simulink model "HaulageOptimizedOperationSimulation_Bea"  (R2026a)
settings: Solver=FixedStepDiscrete  FixedStep=1
libraries: simulink x10
settings Model: Creator=chimb  LastModifiedBy=linuxpc

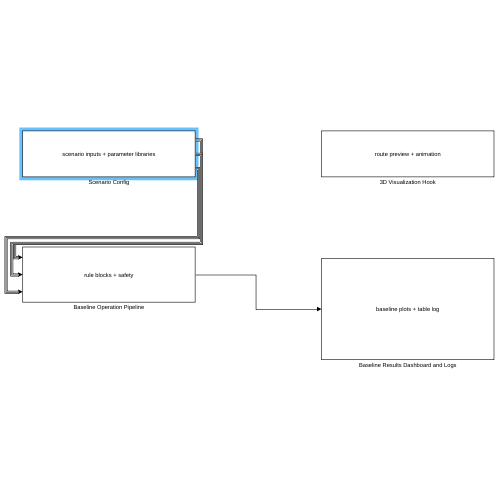
[thumbnail: Simulink's stored preview of the top-level diagram]
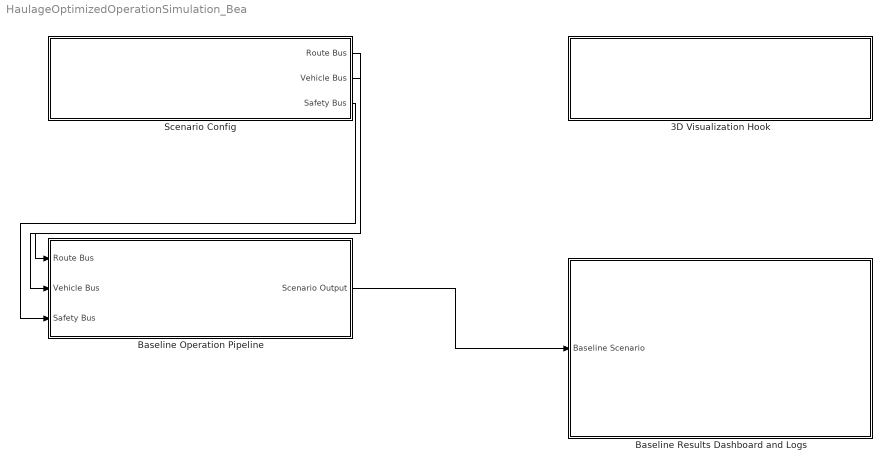
== system HaulageOptimizedOperationSimulation_Bea ==
  3D Visualization Hook : Subsystem
      mask Display: color('black'); disp('route preview + animation')
  Baseline Operation Pipeline : Subsystem
      mask Display: color('black'); disp('rule blocks + safety')
  Baseline Results Dashboard and Logs : Subsystem
      mask Display: color('black'); disp('baseline plots + table log')
  Scenario Config : Subsystem
      mask Display: color('black'); disp('scenario inputs + parameter libraries')
  wires:
  Scenario Config/1(Route Bus) -> Baseline Operation Pipeline/1(Route Bus)
  Scenario Config/2(Vehicle Bus) -> Baseline Operation Pipeline/2(Vehicle Bus)
  Scenario Config/3(Safety Bus) -> Baseline Operation Pipeline/3(Safety Bus)
  Baseline Operation Pipeline/1(Scenario Output) -> Baseline Results Dashboard and Logs/1(Baseline Scenario)

== system HaulageOptimizedOperationSimulation_Bea/3D Visualization Hook ==
  Route 3D Preview Image : Subsystem
      settings: OpenFcn=open('C:/Users/chimb/Documents/Codex/2026-05-20/files-mentioned-by-the-user-paper/haulage_sim_framework/outputs/baseline_operation_route_3d_preview.png')
      mask Display: image(imread('C:/Users/chimb/Documents/Codex/2026-05-20/files-mentioned-by-the-user-paper/haulage_sim_framework/outputs/baseline_operation_route_3d_preview.png'))

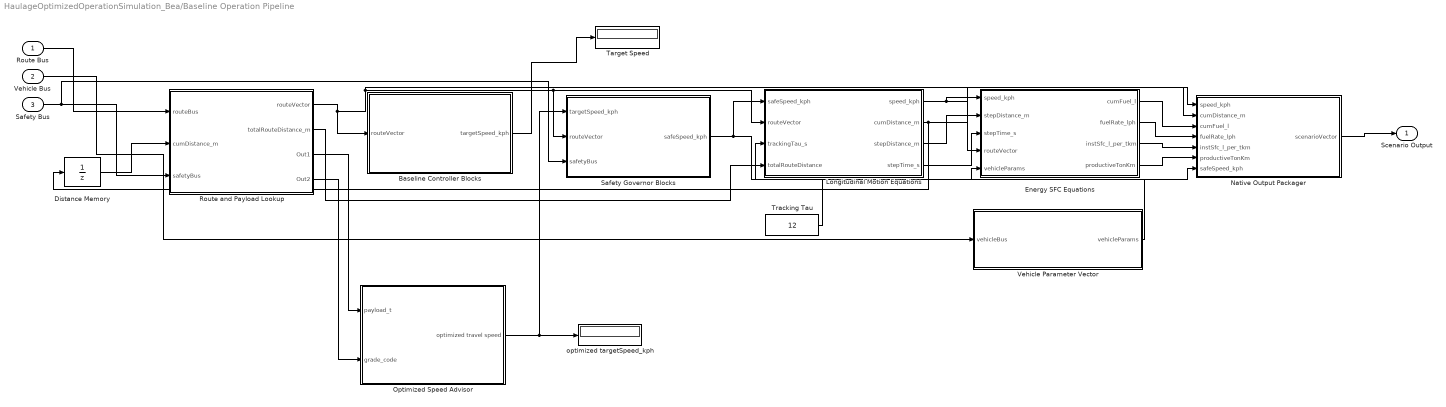
== system HaulageOptimizedOperationSimulation_Bea/Baseline Operation Pipeline ==
  Route Bus : Inport
  Vehicle Bus : Inport  Port=2
  Safety Bus : Inport  Port=3
  Baseline Controller Blocks : Subsystem
      mask Display: color('black'); disp('rule-based speed logic')
  Distance Memory : UnitDelay
  Energy SFC Equations : MATLAB Function  TreatAsAtomicUnit=on
  Longitudinal Motion Equations : MATLAB Function  TreatAsAtomicUnit=on
  Native Output Packager : Subsystem
      mask Display: color('black'); disp('native mux for log vector')
  Optimized Speed Advisor : Subsystem
  Route and Payload Lookup : Subsystem
      mask Display: color('black'); disp('dynamic route lookup tables')
  Safety Governor Blocks : Subsystem
      mask Display: color('black'); disp('speed caps + min/max')
  Target Speed : Display
  Tracking Tau : Constant  Value=12
  Vehicle Parameter Vector : Subsystem
  optimized targetSpeed_kph : Display
  Scenario Output : Outport
  wires:
  Route Bus/1 -> Route and Payload Lookup/1(routeBus)
  Vehicle Bus/1 -> Vehicle Parameter Vector/1(vehicleBus)
  Safety Bus/1 -> Safety Governor Blocks/3(safetyBus), Route and Payload Lookup/3(safetyBus)
  Distance Memory/1 -> Route and Payload Lookup/2(cumDistance_m)
  Route and Payload Lookup/1(routeVector) -> Safety Governor Blocks/2(routeVector), Longitudinal Motion Equations/2(routeVector), Energy SFC Equations/4(routeVector), Baseline Controller Blocks/1(routeVector)
  Baseline Controller Blocks/1(targetSpeed_kph) -> Target Speed/1
  Safety Governor Blocks/1(safeSpeed_kph) -> Longitudinal Motion Equations/1(safeSpeed_kph), Native Output Packager/7(safeSpeed_kph)
  Tracking Tau/1 -> Longitudinal Motion Equations/3(trackingTau_s)
  Route and Payload Lookup/2(totalRouteDistance_m) -> Longitudinal Motion Equations/4(totalRouteDistance)
  Longitudinal Motion Equations/1(speed_kph) -> Energy SFC Equations/1(speed_kph), Native Output Packager/1(speed_kph)
  Longitudinal Motion Equations/3(stepDistance_m) -> Energy SFC Equations/2(stepDistance_m)
  Longitudinal Motion Equations/4(stepTime_s) -> Energy SFC Equations/3(stepTime_s)
  Vehicle Parameter Vector/1(vehicleParams) -> Energy SFC Equations/5(vehicleParams)
  Longitudinal Motion Equations/2(cumDistance_m) -> Native Output Packager/2(cumDistance_m), Distance Memory/1
  Energy SFC Equations/1(cumFuel_l) -> Native Output Packager/3(cumFuel_l)
  Energy SFC Equations/2(fuelRate_lph) -> Native Output Packager/4(fuelRate_lph)
  Energy SFC Equations/3(instSfc_l_per_tkm) -> Native Output Packager/5(instSfc_l_per_tkm)
  Energy SFC Equations/4(productiveTonKm) -> Native Output Packager/6(productiveTonKm)
  Native Output Packager/1(scenarioVector) -> Scenario Output/1
  Route and Payload Lookup/3(Out1) -> Optimized Speed Advisor/1(payload_t)
  Route and Payload Lookup/4(Out2) -> Optimized Speed Advisor/2(grade_code)
  Optimized Speed Advisor/1(optimized travel speed) -> optimized targetSpeed_kph/1, Safety Governor Blocks/1(targetSpeed_kph)

== system HaulageOptimizedOperationSimulation_Bea/Baseline Results Dashboard and Logs ==
  Baseline Scenario : Inport
  Baseline Log : ToWorkspace  VariableName=optimized_operation_log  SaveFormat=Structure With Time  SampleTime=-1
  Baseline Metric Dashboard : Subsystem
      mask Display: color('black'); disp('baseline speed, fuel, SFC, productivity')
  To Workspace : ToWorkspace  VariableName=simout  SaveFormat=Timeseries  SampleTime=-1
  wires:
  Baseline Scenario/1 -> Baseline Log/1, To Workspace/1, Baseline Metric Dashboard/1(Baseline Scenario Vector)

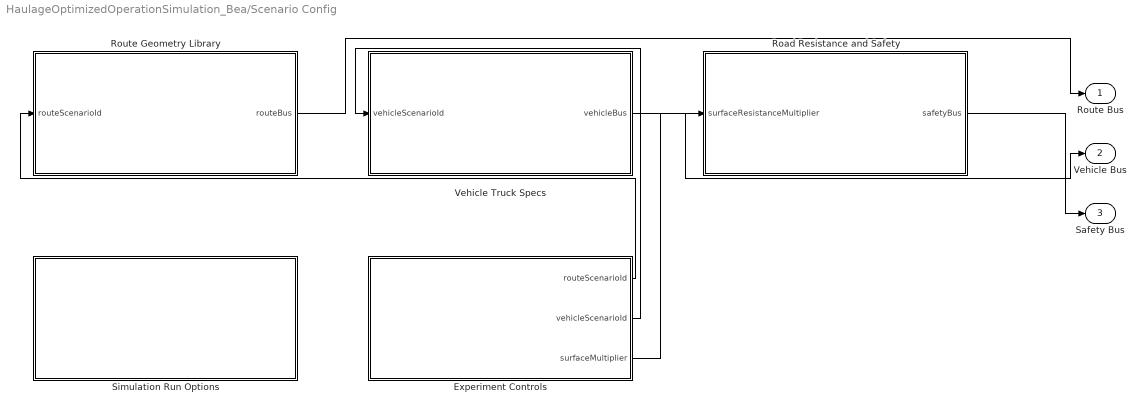
== system HaulageOptimizedOperationSimulation_Bea/Scenario Config ==
  Experiment Controls : Subsystem
      mask Display: color('black'); disp('active experiment selectors')
  Road Resistance and Safety : Subsystem
      mask Display: color('black'); disp('rolling resistance + safety caps')
  Route Geometry Library : Subsystem
      mask Display: color('black'); disp('route segments, grade, limits')
  Simulation Run Options : Subsystem
      mask Display: color('black'); disp('solver, stop time, reporting')
  Vehicle Truck Specs : Subsystem
      mask Display: color('black'); disp('full-scale haul truck specs')
  Route Bus : Outport
  Vehicle Bus : Outport  Port=2
  Safety Bus : Outport  Port=3
  wires:
  Experiment Controls/1(routeScenarioId) -> Route Geometry Library/1(routeScenarioId)
  Experiment Controls/2(vehicleScenarioId) -> Vehicle Truck Specs/1(vehicleScenarioId)
  Experiment Controls/3(surfaceMultiplier) -> Road Resistance and Safety/1(surfaceResistanceMultiplier)
  Route Geometry Library/1(routeBus) -> Route Bus/1
  Vehicle Truck Specs/1(vehicleBus) -> Vehicle Bus/1
  Road Resistance and Safety/1(safetyBus) -> Safety Bus/1

== system HaulageOptimizedOperationSimulation_Bea/3D Visualization Hook/Route 3D Preview Image ==
  Preview Ready Flag : Constant
  Preview Status Display : Display
  wires:
  Preview Ready Flag/1 -> Preview Status Display/1

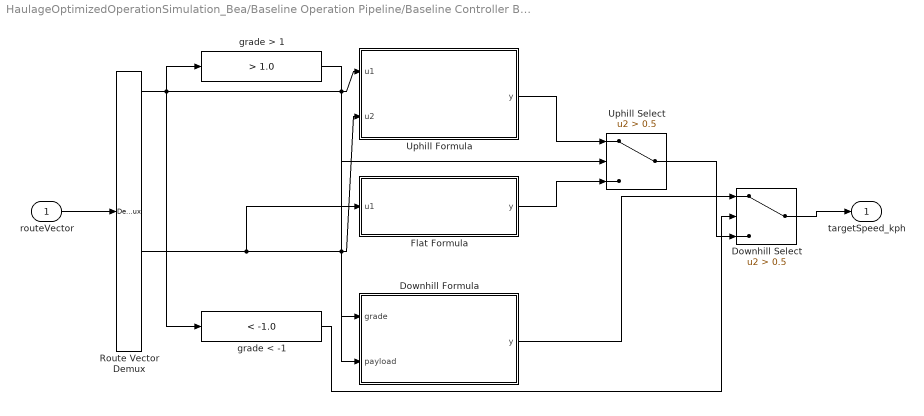
== system HaulageOptimizedOperationSimulation_Bea/Baseline Operation Pipeline/Baseline Controller Blocks ==
  routeVector : Inport
  Downhill Formula : Subsystem
  Downhill Select : Switch  Criteria=u2 > Threshold  Threshold=0.5  SaturateOnIntegerOverflow=off  InputSameDT=off
  Flat Formula : Subsystem
  Route Vector Demux : Demux  Outputs=7
  Uphill Formula : Subsystem
  Uphill Select : Switch  Criteria=u2 > Threshold  Threshold=0.5  SaturateOnIntegerOverflow=off  InputSameDT=off
  grade < -1 : simulink/Logic and Bit Operations/Compare To Constant  relop=<  const=-1.0  OutDataTypeStr=boolean
  grade > 1 : simulink/Logic and Bit Operations/Compare To Constant  relop=>  const=1.0  OutDataTypeStr=boolean
  targetSpeed_kph : Outport
  wires:
  routeVector/1 -> Route Vector Demux/1
  Route Vector Demux/1 -> Uphill Formula/1(u1), Downhill Formula/1(grade), grade > 1/1, grade < -1/1
  Route Vector Demux/5 -> Uphill Formula/2(u2), Downhill Formula/2(payload), Flat Formula/1(u1)
  Uphill Formula/1(y) -> Uphill Select/1
  grade > 1/1 -> Uphill Select/2
  Flat Formula/1(y) -> Uphill Select/3
  Downhill Formula/1(y) -> Downhill Select/1
  grade < -1/1 -> Downhill Select/2
  Uphill Select/1 -> Downhill Select/3
  Downhill Select/1 -> targetSpeed_kph/1

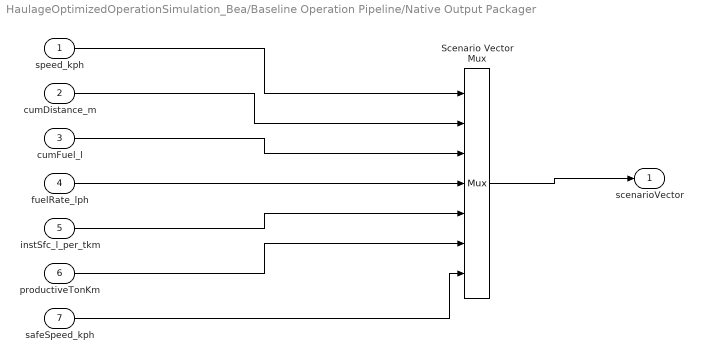
== system HaulageOptimizedOperationSimulation_Bea/Baseline Operation Pipeline/Native Output Packager ==
  speed_kph : Inport
  cumDistance_m : Inport  Port=2
  cumFuel_l : Inport  Port=3
  fuelRate_lph : Inport  Port=4
  instSfc_l_per_tkm : Inport  Port=5
  productiveTonKm : Inport  Port=6
  safeSpeed_kph : Inport  Port=7
  Scenario Vector Mux : Mux  Inputs=7
  scenarioVector : Outport
  wires:
  speed_kph/1 -> Scenario Vector Mux/1
  cumDistance_m/1 -> Scenario Vector Mux/2
  cumFuel_l/1 -> Scenario Vector Mux/3
  fuelRate_lph/1 -> Scenario Vector Mux/4
  instSfc_l_per_tkm/1 -> Scenario Vector Mux/5
  productiveTonKm/1 -> Scenario Vector Mux/6
  safeSpeed_kph/1 -> Scenario Vector Mux/7
  Scenario Vector Mux/1 -> scenarioVector/1

== system HaulageOptimizedOperationSimulation_Bea/Baseline Operation Pipeline/Optimized Speed Advisor ==
  note: opt_speed_kph column from the ml_speed_policy_table.csv
      | For our current open-pit route, the truck is:
      | loaded at 279 t on segments S1-S5;
      | empty at 0 t on segments S6-S8.
  payload_t : Inport
  grade_code : Inport  Port=2
  Downhill : MATLAB Function  TreatAsAtomicUnit=on
  Flat : MATLAB Function  TreatAsAtomicUnit=on
  Multiport Switch : MultiPortSwitch  SaturateOnIntegerOverflow=off  InputSameDT=off
  Uphill : MATLAB Function  TreatAsAtomicUnit=on
  optimized travel speed : Outport
  wires:
  payload_t/1 -> Downhill/1(u), Flat/1(u), Uphill/1(u)
  Uphill/1(y) -> Multiport Switch/2
  Flat/1(y) -> Multiport Switch/3
  Downhill/1(y) -> Multiport Switch/4
  grade_code/1 -> Multiport Switch/1
  Multiport Switch/1 -> optimized travel speed/1

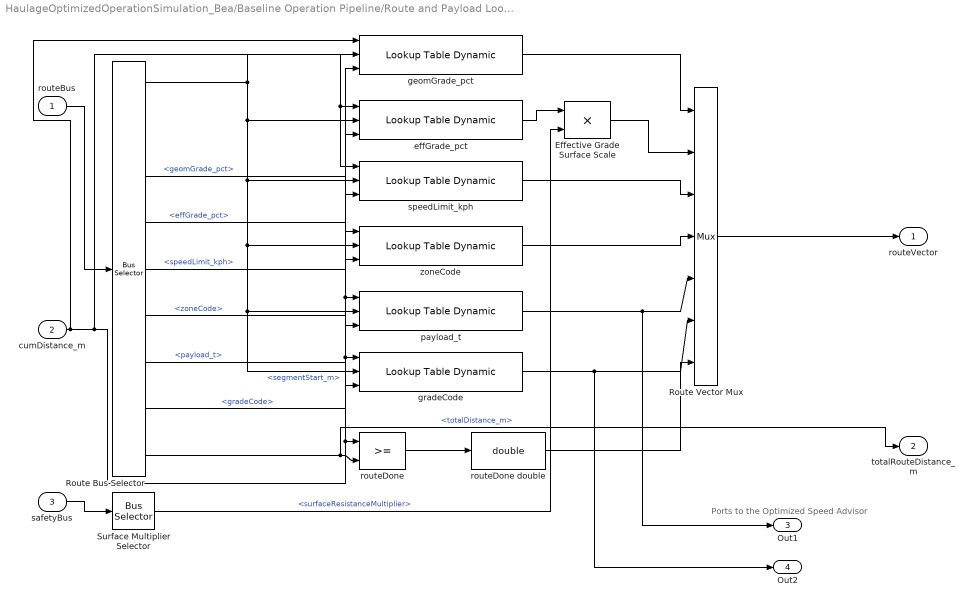
== system HaulageOptimizedOperationSimulation_Bea/Baseline Operation Pipeline/Route and Payload Lookup ==
  note: Ports to the Optimized Speed Advisor
  routeBus : Inport
  cumDistance_m : Inport  Port=2
  safetyBus : Inport  Port=3
  Effective Grade Surface Scale : Product
  Route Bus Selector : BusSelector  OutputSignals=segmentStart_m,segmentEnd_m,geomGrade_pct,effGrade_pct,speedLimit_kph,zoneCode,payload_t,gradeCode,totalDistance_m
  Route Vector Mux : Mux  Inputs=7
  Surface Multiplier Selector : BusSelector  OutputSignals=surfaceResistanceMultiplier
  effGrade_pct : simulink/Lookup Tables/Lookup Table Dynamic  LookUpMeth=Use Input Below  OutDataType=fixdt('double')  OutScaling=[]  OutputDataTypeScalingMode=Specify via dialog  OutDataTypeStr=double  DoSatur=off
  geomGrade_pct : simulink/Lookup Tables/Lookup Table Dynamic  LookUpMeth=Use Input Below  OutDataType=fixdt('double')  OutScaling=[]  OutputDataTypeScalingMode=Specify via dialog  OutDataTypeStr=double  DoSatur=off
  gradeCode : simulink/Lookup Tables/Lookup Table Dynamic  LookUpMeth=Use Input Below  OutDataType=fixdt('double')  OutScaling=[]  OutputDataTypeScalingMode=Specify via dialog  OutDataTypeStr=double  DoSatur=off
  payload_t : simulink/Lookup Tables/Lookup Table Dynamic  LookUpMeth=Use Input Below  OutDataType=fixdt('double')  OutScaling=[]  OutputDataTypeScalingMode=Specify via dialog  OutDataTypeStr=double  DoSatur=off
  routeDone : RelationalOperator  OutDataTypeStr=boolean  RndMeth=Simplest  InputSameDT=off
  routeDone double : DataTypeConversion  OutDataTypeStr=double  SaturateOnIntegerOverflow=off  RndMeth=Floor
  speedLimit_kph : simulink/Lookup Tables/Lookup Table Dynamic  LookUpMeth=Use Input Below  OutDataType=fixdt('double')  OutScaling=[]  OutputDataTypeScalingMode=Specify via dialog  OutDataTypeStr=double  DoSatur=off
  zoneCode : simulink/Lookup Tables/Lookup Table Dynamic  LookUpMeth=Use Input Below  OutDataType=fixdt('double')  OutScaling=[]  OutputDataTypeScalingMode=Specify via dialog  OutDataTypeStr=double  DoSatur=off
  routeVector : Outport
  totalRouteDistance_m : Outport  Port=2
  Out1 : Outport  Port=3
  Out2 : Outport  Port=4
  wires:
  routeBus/1 -> Route Bus Selector/1
  safetyBus/1 -> Surface Multiplier Selector/1
  cumDistance_m/1 -> zoneCode/1, payload_t/1, gradeCode/1, routeDone/1, effGrade_pct/1, speedLimit_kph/1, geomGrade_pct/1
  Route Bus Selector/1 -> payload_t/2, gradeCode/2, zoneCode/2, speedLimit_kph/2, effGrade_pct/2, geomGrade_pct/2  "<segmentStart_m>"
  Route Bus Selector/3 -> geomGrade_pct/3  "<geomGrade_pct>"
  Route Bus Selector/4 -> effGrade_pct/3  "<effGrade_pct>"
  Route Bus Selector/5 -> speedLimit_kph/3  "<speedLimit_kph>"
  Route Bus Selector/6 -> zoneCode/3  "<zoneCode>"
  Route Bus Selector/7 -> payload_t/3  "<payload_t>"
  Route Bus Selector/8 -> gradeCode/3  "<gradeCode>"
  effGrade_pct/1 -> Effective Grade Surface Scale/1
  Surface Multiplier Selector/1 -> Effective Grade Surface Scale/2  "<surfaceResistanceMultiplier>"
  Route Bus Selector/9 -> routeDone/2, totalRouteDistance_m/1  "<totalDistance_m>"
  routeDone/1 -> routeDone double/1
  geomGrade_pct/1 -> Route Vector Mux/1
  Effective Grade Surface Scale/1 -> Route Vector Mux/2
  speedLimit_kph/1 -> Route Vector Mux/3
  zoneCode/1 -> Route Vector Mux/4
  gradeCode/1 -> Out2/1, Route Vector Mux/6
  routeDone double/1 -> Route Vector Mux/7
  Route Vector Mux/1 -> routeVector/1
  payload_t/1 -> Out1/1, Route Vector Mux/5

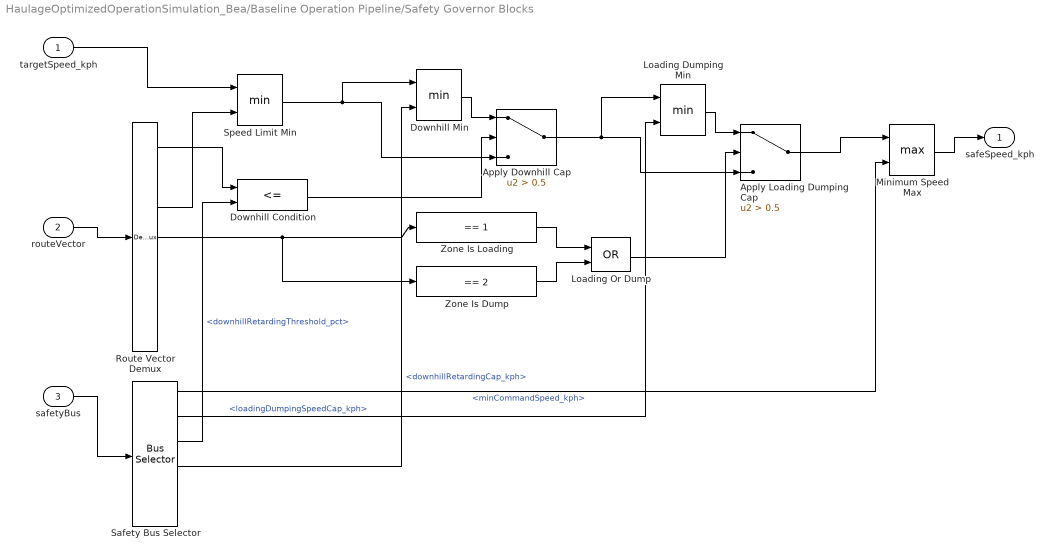
== system HaulageOptimizedOperationSimulation_Bea/Baseline Operation Pipeline/Safety Governor Blocks ==
  targetSpeed_kph : Inport
  routeVector : Inport  Port=2
  safetyBus : Inport  Port=3
  Apply Downhill Cap : Switch  Criteria=u2 > Threshold  Threshold=0.5  SaturateOnIntegerOverflow=off  InputSameDT=off
  Apply Loading Dumping Cap : Switch  Criteria=u2 > Threshold  Threshold=0.5  SaturateOnIntegerOverflow=off  InputSameDT=off
  Downhill Condition : RelationalOperator  Operator=<=  OutDataTypeStr=boolean  RndMeth=Simplest  InputSameDT=off
  Downhill Min : MinMax  Inputs=2
  Loading Dumping Min : MinMax  Inputs=2
  Loading Or Dump : Logic  Operator=OR  AllPortsSameDT=off  OutDataTypeStr=boolean
  Minimum Speed Max : MinMax  Function=max  Inputs=2
  Route Vector Demux : Demux  Outputs=7
  Safety Bus Selector : BusSelector  OutputSignals=minCommandSpeed_kph,loadingDumpingSpeedCap_kph,downhillRetardingThreshold_pct,downhillRetardingCap_kph,maxOperatingSpeed_kph,surfaceResistanceMultiplier
  Speed Limit Min : MinMax  Inputs=2
  Zone Is Dump : simulink/Logic and Bit Operations/Compare To Constant  relop===  const=2  OutDataTypeStr=boolean
  Zone Is Loading : simulink/Logic and Bit Operations/Compare To Constant  relop===  const=1  OutDataTypeStr=boolean
  safeSpeed_kph : Outport
  wires:
  routeVector/1 -> Route Vector Demux/1
  safetyBus/1 -> Safety Bus Selector/1
  targetSpeed_kph/1 -> Speed Limit Min/1
  Route Vector Demux/3 -> Speed Limit Min/2
  Route Vector Demux/1 -> Downhill Condition/1
  Safety Bus Selector/3 -> Downhill Condition/2  "<downhillRetardingThreshold_pct>"
  Speed Limit Min/1 -> Downhill Min/1, Apply Downhill Cap/3
  Safety Bus Selector/4 -> Downhill Min/2  "<downhillRetardingCap_kph>"
  Downhill Min/1 -> Apply Downhill Cap/1
  Downhill Condition/1 -> Apply Downhill Cap/2
  Route Vector Demux/4 -> Zone Is Loading/1, Zone Is Dump/1
  Zone Is Loading/1 -> Loading Or Dump/1
  Zone Is Dump/1 -> Loading Or Dump/2
  Apply Downhill Cap/1 -> Loading Dumping Min/1, Apply Loading Dumping Cap/3
  Safety Bus Selector/2 -> Loading Dumping Min/2  "<loadingDumpingSpeedCap_kph>"
  Loading Dumping Min/1 -> Apply Loading Dumping Cap/1
  Loading Or Dump/1 -> Apply Loading Dumping Cap/2
  Apply Loading Dumping Cap/1 -> Minimum Speed Max/1
  Safety Bus Selector/1 -> Minimum Speed Max/2  "<minCommandSpeed_kph>"
  Minimum Speed Max/1 -> safeSpeed_kph/1

== system HaulageOptimizedOperationSimulation_Bea/Baseline Operation Pipeline/Vehicle Parameter Vector ==
  vehicleBus : Inport
  Vehicle Bus Selector : BusSelector  OutputSignals=emptyMass_kg,idleFuelRate_lph,maxFuelRate_lph,frontalArea_m2,dragCoefficient,drivetrainEfficiency
  Vehicle Params Mux : Mux  Inputs=6
  vehicleParams : Outport
  wires:
  vehicleBus/1 -> Vehicle Bus Selector/1
  Vehicle Bus Selector/1 -> Vehicle Params Mux/1  "<emptyMass_kg>"
  Vehicle Bus Selector/2 -> Vehicle Params Mux/2  "<idleFuelRate_lph>"
  Vehicle Bus Selector/3 -> Vehicle Params Mux/3  "<maxFuelRate_lph>"
  Vehicle Bus Selector/4 -> Vehicle Params Mux/4  "<frontalArea_m2>"
  Vehicle Bus Selector/5 -> Vehicle Params Mux/5  "<dragCoefficient>"
  Vehicle Bus Selector/6 -> Vehicle Params Mux/6  "<drivetrainEfficiency>"
  Vehicle Params Mux/1 -> vehicleParams/1

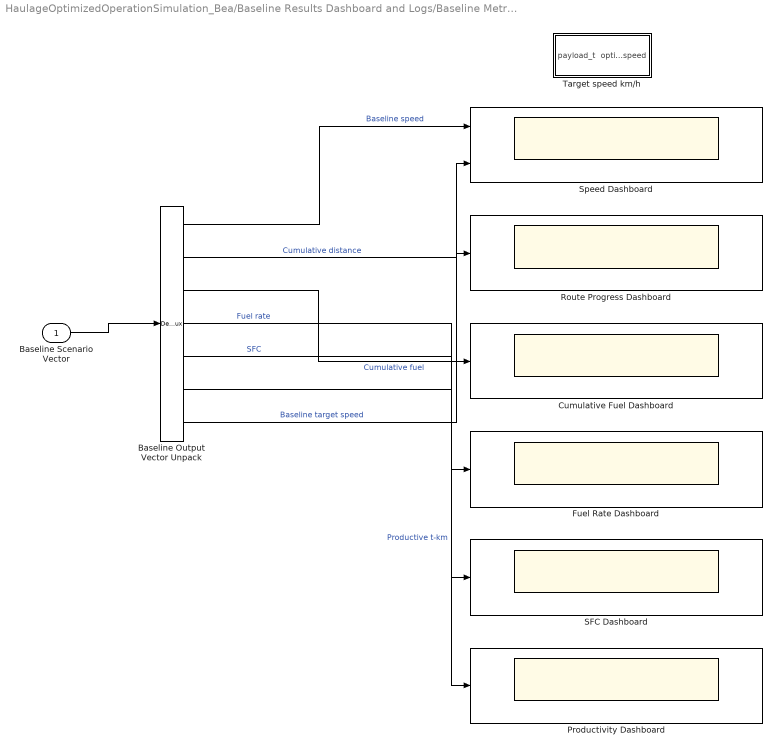
== system HaulageOptimizedOperationSimulation_Bea/Baseline Results Dashboard and Logs/Baseline Metric Dashboard ==
  Baseline Scenario Vector : Inport
  Baseline Output Vector Unpack : Demux  Outputs=7
  Cumulative Fuel Dashboard : Scope
      settings: Title=Baseline Cumulative Fuel Use  ActiveDisplayYMinimum=-0.7369719012317395  ActiveDisplayYMaximum=6.6567683881931847  YLabel=Fuel (L)
  Fuel Rate Dashboard : Scope
      settings: Title=Baseline Fuel Rate Along Cycle  ActiveDisplayYMinimum=-3.9999999999999982  ActiveDisplayYMaximum=106  YLabel=Fuel rate (L/h)
  Productivity Dashboard : Scope
      settings: Title=Baseline Productive Haulage Work  ActiveDisplayYMinimum=-27.831999586920773  ActiveDisplayYMaximum=251.262996282287  YLabel=Productive work (t-km)
  Route Progress Dashboard : Scope
      settings: Title=Baseline Route Progress  ActiveDisplayYMinimum=-192.18749999999994  ActiveDisplayYMaximum=1732.4652777777778  YLabel=Cumulative distance (m)
  SFC Dashboard : Scope
      settings: Title=Baseline Specific Fuel Consumption  ActiveDisplayYMinimum=-0.00247472099881277  ActiveDisplayYMaximum=0.036217610604932046  YLabel=SFC (L/t-km)
  Speed Dashboard : Scope  NumInputPorts=2
      settings: Title=Baseline Speed and Command  ActiveDisplayYMinimum=-1.1249999999999998  ActiveDisplayYMaximum=20.125  YLabel=Speed (km/h)
  Target speed km/h : Subsystem
  wires:
  Baseline Scenario Vector/1 -> Baseline Output Vector Unpack/1
  Baseline Output Vector Unpack/1 -> Speed Dashboard/1  "Baseline speed"
  Baseline Output Vector Unpack/7 -> Speed Dashboard/2  "Baseline target speed"
  Baseline Output Vector Unpack/2 -> Route Progress Dashboard/1  "Cumulative distance"
  Baseline Output Vector Unpack/3 -> Cumulative Fuel Dashboard/1  "Cumulative fuel"
  Baseline Output Vector Unpack/4 -> Fuel Rate Dashboard/1  "Fuel rate"
  Baseline Output Vector Unpack/5 -> SFC Dashboard/1  "SFC"
  Baseline Output Vector Unpack/6 -> Productivity Dashboard/1  "Productive t-km"

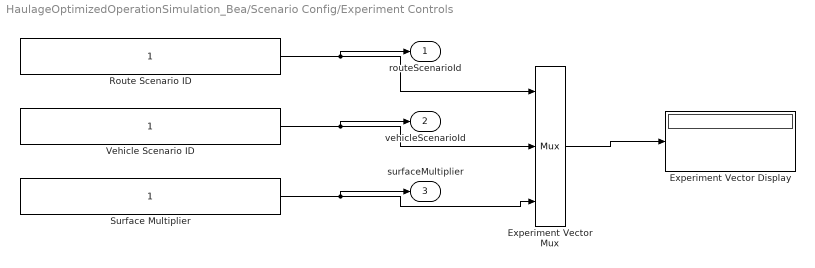
== system HaulageOptimizedOperationSimulation_Bea/Scenario Config/Experiment Controls ==
  Experiment Vector Display : Display
  Experiment Vector Mux : Mux  Inputs=3
  Route Scenario ID : Constant
  Surface Multiplier : Constant
  Vehicle Scenario ID : Constant
  routeScenarioId : Outport
  vehicleScenarioId : Outport  Port=2
  surfaceMultiplier : Outport  Port=3
  wires:
  Route Scenario ID/1 -> Experiment Vector Mux/1, routeScenarioId/1
  Vehicle Scenario ID/1 -> Experiment Vector Mux/2, vehicleScenarioId/1
  Surface Multiplier/1 -> Experiment Vector Mux/3, surfaceMultiplier/1
  Experiment Vector Mux/1 -> Experiment Vector Display/1

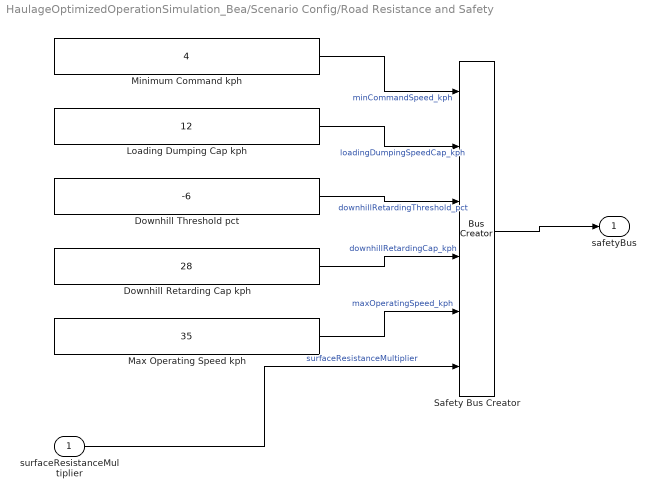
== system HaulageOptimizedOperationSimulation_Bea/Scenario Config/Road Resistance and Safety ==
  surfaceResistanceMultiplier : Inport
  Downhill Retarding Cap kph : Constant  Value=28
  Downhill Threshold pct : Constant  Value=-6
  Loading Dumping Cap kph : Constant  Value=12
  Max Operating Speed kph : Constant  Value=35
  Minimum Command kph : Constant  Value=4
  Safety Bus Creator : BusCreator  Inputs=6
  safetyBus : Outport
  wires:
  Minimum Command kph/1 -> Safety Bus Creator/1  "minCommandSpeed_kph"
  Loading Dumping Cap kph/1 -> Safety Bus Creator/2  "loadingDumpingSpeedCap_kph"
  Downhill Threshold pct/1 -> Safety Bus Creator/3  "downhillRetardingThreshold_pct"
  Downhill Retarding Cap kph/1 -> Safety Bus Creator/4  "downhillRetardingCap_kph"
  Max Operating Speed kph/1 -> Safety Bus Creator/5  "maxOperatingSpeed_kph"
  surfaceResistanceMultiplier/1 -> Safety Bus Creator/6  "surfaceResistanceMultiplier"
  Safety Bus Creator/1 -> safetyBus/1

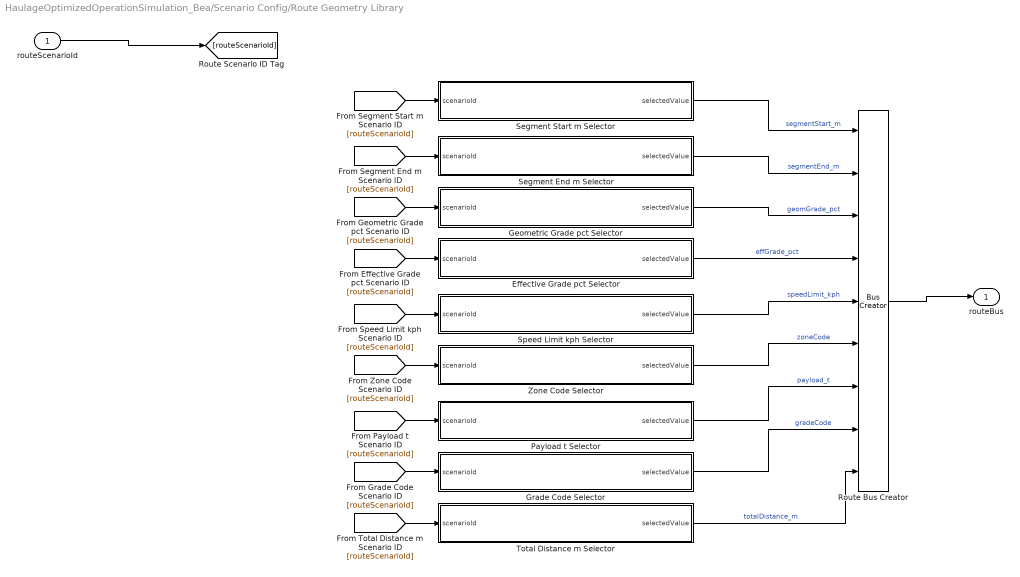
== system HaulageOptimizedOperationSimulation_Bea/Scenario Config/Route Geometry Library ==
  routeScenarioId : Inport
  Effective Grade pct Selector : Subsystem
      mask Display: color('black'); disp('editable effective grade pct scenario selector')
  Geometric Grade pct Selector : Subsystem
      mask Display: color('black'); disp('editable geometric grade pct scenario selector')
  Grade Code Selector : Subsystem
      mask Display: color('black'); disp('editable grade code scenario selector')
  Payload t Selector : Subsystem
      mask Display: color('black'); disp('editable payload t scenario selector')
  Route Bus Creator : BusCreator  Inputs=9
  Segment End m Selector : Subsystem
      mask Display: color('black'); disp('editable segment end m scenario selector')
  Segment Start m Selector : Subsystem
      mask Display: color('black'); disp('editable segment start m scenario selector')
  Speed Limit kph Selector : Subsystem
      mask Display: color('black'); disp('editable speed limit kph scenario selector')
  Total Distance m Selector : Subsystem
      mask Display: color('black'); disp('editable total distance m scenario selector')
  Zone Code Selector : Subsystem
      mask Display: color('black'); disp('editable zone code scenario selector')
  routeBus : Outport
  wires:
  routeScenarioId/1 -> [routeScenarioId]
  [routeScenarioId] -> Segment Start m Selector/1(scenarioId)
  [routeScenarioId] -> Segment End m Selector/1(scenarioId)
  [routeScenarioId] -> Geometric Grade pct Selector/1(scenarioId)
  [routeScenarioId] -> Effective Grade pct Selector/1(scenarioId)
  [routeScenarioId] -> Speed Limit kph Selector/1(scenarioId)
  [routeScenarioId] -> Zone Code Selector/1(scenarioId)
  [routeScenarioId] -> Payload t Selector/1(scenarioId)
  [routeScenarioId] -> Grade Code Selector/1(scenarioId)
  [routeScenarioId] -> Total Distance m Selector/1(scenarioId)
  Segment Start m Selector/1(selectedValue) -> Route Bus Creator/1  "segmentStart_m"
  Segment End m Selector/1(selectedValue) -> Route Bus Creator/2  "segmentEnd_m"
  Geometric Grade pct Selector/1(selectedValue) -> Route Bus Creator/3  "geomGrade_pct"
  Effective Grade pct Selector/1(selectedValue) -> Route Bus Creator/4  "effGrade_pct"
  Speed Limit kph Selector/1(selectedValue) -> Route Bus Creator/5  "speedLimit_kph"
  Zone Code Selector/1(selectedValue) -> Route Bus Creator/6  "zoneCode"
  Payload t Selector/1(selectedValue) -> Route Bus Creator/7  "payload_t"
  Grade Code Selector/1(selectedValue) -> Route Bus Creator/8  "gradeCode"
  Total Distance m Selector/1(selectedValue) -> Route Bus Creator/9  "totalDistance_m"
  Route Bus Creator/1 -> routeBus/1

== system HaulageOptimizedOperationSimulation_Bea/Scenario Config/Simulation Run Options ==
  Baseline Tracking Tau s : Constant  Value=12
  Clock Display : Display
  Fixed Step dt s : Constant
  Output Vector Width : Constant  Value=7
  Simulation Clock : Clock
  Stop Time s : Constant  Value=1400
  wires:
  Simulation Clock/1 -> Clock Display/1

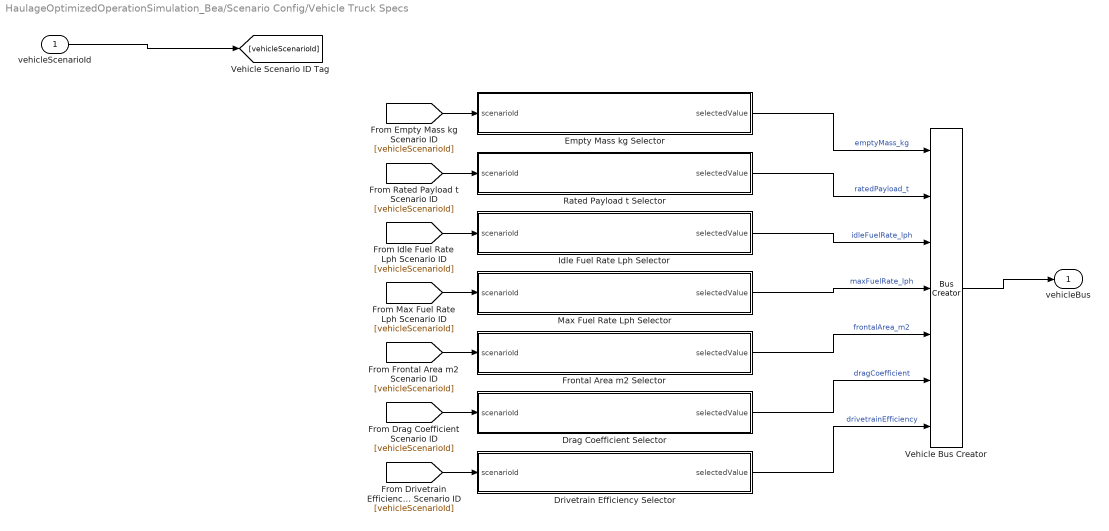
== system HaulageOptimizedOperationSimulation_Bea/Scenario Config/Vehicle Truck Specs ==
  vehicleScenarioId : Inport
  Drag Coefficient Selector : Subsystem
      mask Display: color('black'); disp('editable drag coefficient scenario selector')
  Drivetrain Efficiency Selector : Subsystem
      mask Display: color('black'); disp('editable drivetrain efficiency scenario selector')
  Empty Mass kg Selector : Subsystem
      mask Display: color('black'); disp('editable empty mass kg scenario selector')
  Frontal Area m2 Selector : Subsystem
      mask Display: color('black'); disp('editable frontal area m2 scenario selector')
  Idle Fuel Rate Lph Selector : Subsystem
      mask Display: color('black'); disp('editable idle fuel rate lph scenario selector')
  Max Fuel Rate Lph Selector : Subsystem
      mask Display: color('black'); disp('editable max fuel rate lph scenario selector')
  Rated Payload t Selector : Subsystem
      mask Display: color('black'); disp('editable rated payload t scenario selector')
  Vehicle Bus Creator : BusCreator  Inputs=7
  vehicleBus : Outport
  wires:
  vehicleScenarioId/1 -> [vehicleScenarioId]
  [vehicleScenarioId] -> Empty Mass kg Selector/1(scenarioId)
  [vehicleScenarioId] -> Rated Payload t Selector/1(scenarioId)
  [vehicleScenarioId] -> Idle Fuel Rate Lph Selector/1(scenarioId)
  [vehicleScenarioId] -> Max Fuel Rate Lph Selector/1(scenarioId)
  [vehicleScenarioId] -> Frontal Area m2 Selector/1(scenarioId)
  [vehicleScenarioId] -> Drag Coefficient Selector/1(scenarioId)
  [vehicleScenarioId] -> Drivetrain Efficiency Selector/1(scenarioId)
  Empty Mass kg Selector/1(selectedValue) -> Vehicle Bus Creator/1  "emptyMass_kg"
  Rated Payload t Selector/1(selectedValue) -> Vehicle Bus Creator/2  "ratedPayload_t"
  Idle Fuel Rate Lph Selector/1(selectedValue) -> Vehicle Bus Creator/3  "idleFuelRate_lph"
  Max Fuel Rate Lph Selector/1(selectedValue) -> Vehicle Bus Creator/4  "maxFuelRate_lph"
  Frontal Area m2 Selector/1(selectedValue) -> Vehicle Bus Creator/5  "frontalArea_m2"
  Drag Coefficient Selector/1(selectedValue) -> Vehicle Bus Creator/6  "dragCoefficient"
  Drivetrain Efficiency Selector/1(selectedValue) -> Vehicle Bus Creator/7  "drivetrainEfficiency"
  Vehicle Bus Creator/1 -> vehicleBus/1

== system HaulageOptimizedOperationSimulation_Bea/Baseline Operation Pipeline/Baseline Controller Blocks/Downhill Formula ==
  grade : Inport
  payload : Inport  Port=2
  abs grade : Abs  SaturateOnIntegerOverflow=off
  grade gain : Gain  Gain=0.20
  offset : Constant  Value=22
  payload gain : Gain  Gain=-0.003
  sum : Sum  Inputs=+++
  y : Outport
  wires:
  grade/1 -> abs grade/1
  abs grade/1 -> grade gain/1
  payload/1 -> payload gain/1
  grade gain/1 -> sum/1
  payload gain/1 -> sum/2
  offset/1 -> sum/3
  sum/1 -> y/1

== system HaulageOptimizedOperationSimulation_Bea/Baseline Operation Pipeline/Baseline Controller Blocks/Flat Formula ==
  u1 : Inport
  gain1 : Gain  Gain=-0.005
  offset : Constant  Value=26
  sum : Sum
  y : Outport
  wires:
  u1/1 -> gain1/1
  gain1/1 -> sum/1
  offset/1 -> sum/2
  sum/1 -> y/1

== system HaulageOptimizedOperationSimulation_Bea/Baseline Operation Pipeline/Baseline Controller Blocks/Uphill Formula ==
  u1 : Inport
  u2 : Inport  Port=2
  gain1 : Gain  Gain=-0.9
  gain2 : Gain  Gain=-0.01
  offset : Constant  Value=22
  sum : Sum  Inputs=+++
  y : Outport
  wires:
  u1/1 -> gain1/1
  u2/1 -> gain2/1
  gain1/1 -> sum/1
  gain2/1 -> sum/2
  offset/1 -> sum/3
  sum/1 -> y/1

== system HaulageOptimizedOperationSimulation_Bea/Baseline Results Dashboard and Logs/Baseline Metric Dashboard/Target speed km//h ==
  payload_t : Inport
  Uphill : MATLAB Function  TreatAsAtomicUnit=on
  optimized travel speed : Outport

== system HaulageOptimizedOperationSimulation_Bea/Scenario Config/Route Geometry Library/Effective Grade pct Selector ==
  scenarioId : Inport
  Effective Grade pct lab_track : Constant  Value=[1.5 5.8 10 1.5 1.5 1.5 -4.2 1.5]
  Effective Grade pct open_pit : Constant  Value=[3 9 11 2.2 4.2 1.8 -4.2 0.9]
  Effective Grade pct underground : Constant  Value=[0.6 -4.8 3.3 3 3 10.1 3.6 3.6]
  Select Effective Grade pct : MultiPortSwitch  SaturateOnIntegerOverflow=off  InputSameDT=off
  selectedValue : Outport
  wires:
  scenarioId/1 -> [routeScenarioId]
  [routeScenarioId] -> Select Effective Grade pct/1
  Effective Grade pct open_pit/1 -> Select Effective Grade pct/2
  Effective Grade pct underground/1 -> Select Effective Grade pct/3
  Effective Grade pct lab_track/1 -> Select Effective Grade pct/4
  Select Effective Grade pct/1 -> selectedValue/1

== system HaulageOptimizedOperationSimulation_Bea/Scenario Config/Route Geometry Library/Geometric Grade pct Selector ==
  scenarioId : Inport
  Geometric Grade pct lab_track : Constant  Value=[0 4 8 0 0 0 -6 0]
  Geometric Grade pct open_pit : Constant  Value=[1 6.5 8 0.2 2 -0.2 -7 -1.5]
  Geometric Grade pct underground : Constant  Value=[-2 -8 0.5 0 0.2 7 1 1]
  Select Geometric Grade pct : MultiPortSwitch  SaturateOnIntegerOverflow=off  InputSameDT=off
  selectedValue : Outport
  wires:
  scenarioId/1 -> [routeScenarioId]
  [routeScenarioId] -> Select Geometric Grade pct/1
  Geometric Grade pct open_pit/1 -> Select Geometric Grade pct/2
  Geometric Grade pct underground/1 -> Select Geometric Grade pct/3
  Geometric Grade pct lab_track/1 -> Select Geometric Grade pct/4
  Select Geometric Grade pct/1 -> selectedValue/1

== system HaulageOptimizedOperationSimulation_Bea/Scenario Config/Route Geometry Library/Grade Code Selector ==
  scenarioId : Inport
  Grade Code lab_track : Constant  Value=[2 1 1 2 2 2 3 2]
  Grade Code open_pit : Constant  Value=[2 1 1 2 1 2 3 3]
  Grade Code underground : Constant  Value=[3 3 2 2 2 1 2 2]
  Select Grade Code : MultiPortSwitch  SaturateOnIntegerOverflow=off  InputSameDT=off
  selectedValue : Outport
  wires:
  scenarioId/1 -> [routeScenarioId]
  [routeScenarioId] -> Select Grade Code/1
  Grade Code open_pit/1 -> Select Grade Code/2
  Grade Code underground/1 -> Select Grade Code/3
  Grade Code lab_track/1 -> Select Grade Code/4
  Select Grade Code/1 -> selectedValue/1

== system HaulageOptimizedOperationSimulation_Bea/Scenario Config/Route Geometry Library/Payload t Selector ==
  scenarioId : Inport
  Payload t lab_track : Constant  Value=[279 279 279 279 279 0 0 0]
  Payload t open_pit : Constant  Value=[279 279 279 279 279 0 0 0]
  Payload t underground : Constant  Value=[279 279 279 279 0 0 0 0]
  Select Payload t : MultiPortSwitch  SaturateOnIntegerOverflow=off  InputSameDT=off
  selectedValue : Outport
  wires:
  scenarioId/1 -> [routeScenarioId]
  [routeScenarioId] -> Select Payload t/1
  Payload t open_pit/1 -> Select Payload t/2
  Payload t underground/1 -> Select Payload t/3
  Payload t lab_track/1 -> Select Payload t/4
  Select Payload t/1 -> selectedValue/1

== system HaulageOptimizedOperationSimulation_Bea/Scenario Config/Route Geometry Library/Segment End m Selector ==
  scenarioId : Inport
  Segment End m lab_track : Constant  Value=[2 5 8 10.5 12 15 19 21]
  Segment End m open_pit : Constant  Value=[180 700 1340 1760 1980 2480 3300 3560]
  Segment End m underground : Constant  Value=[120 480 720 800 1100 1440 1540 1540]
  Select Segment End m : MultiPortSwitch  SaturateOnIntegerOverflow=off  InputSameDT=off
  selectedValue : Outport
  wires:
  scenarioId/1 -> [routeScenarioId]
  [routeScenarioId] -> Select Segment End m/1
  Segment End m open_pit/1 -> Select Segment End m/2
  Segment End m underground/1 -> Select Segment End m/3
  Segment End m lab_track/1 -> Select Segment End m/4
  Select Segment End m/1 -> selectedValue/1

== system HaulageOptimizedOperationSimulation_Bea/Scenario Config/Route Geometry Library/Segment Start m Selector ==
  scenarioId : Inport
  Segment Start m lab_track : Constant  Value=[0 2 5 8 10.5 12 15 19]
  Segment Start m open_pit : Constant  Value=[0 180 700 1340 1760 1980 2480 3300]
  Segment Start m underground : Constant  Value=[0 120 480 720 800 1100 1440 1541]
  Select Segment Start m : MultiPortSwitch  SaturateOnIntegerOverflow=off  InputSameDT=off
  selectedValue : Outport
  wires:
  scenarioId/1 -> [routeScenarioId]
  [routeScenarioId] -> Select Segment Start m/1
  Segment Start m open_pit/1 -> Select Segment Start m/2
  Segment Start m underground/1 -> Select Segment Start m/3
  Segment Start m lab_track/1 -> Select Segment Start m/4
  Select Segment Start m/1 -> selectedValue/1

== system HaulageOptimizedOperationSimulation_Bea/Scenario Config/Route Geometry Library/Speed Limit kph Selector ==
  scenarioId : Inport
  Select Speed Limit kph : MultiPortSwitch  SaturateOnIntegerOverflow=off  InputSameDT=off
  Speed Limit kph lab_track : Constant  Value=[1.5 1.2 1 1.8 1 1.8 1.2 1]
  Speed Limit kph open_pit : Constant  Value=[18 28 25 35 16 35 28 16]
  Speed Limit kph underground : Constant  Value=[12 18 16 8 16 14 12 12]
  selectedValue : Outport
  wires:
  scenarioId/1 -> [routeScenarioId]
  [routeScenarioId] -> Select Speed Limit kph/1
  Speed Limit kph open_pit/1 -> Select Speed Limit kph/2
  Speed Limit kph underground/1 -> Select Speed Limit kph/3
  Speed Limit kph lab_track/1 -> Select Speed Limit kph/4
  Select Speed Limit kph/1 -> selectedValue/1

== system HaulageOptimizedOperationSimulation_Bea/Scenario Config/Route Geometry Library/Total Distance m Selector ==
  scenarioId : Inport
  Select Total Distance m : MultiPortSwitch  SaturateOnIntegerOverflow=off  InputSameDT=off
  Total Distance m lab_track : Constant  Value=21
  Total Distance m open_pit : Constant  Value=3560
  Total Distance m underground : Constant  Value=1540
  selectedValue : Outport
  wires:
  scenarioId/1 -> [routeScenarioId]
  [routeScenarioId] -> Select Total Distance m/1
  Total Distance m open_pit/1 -> Select Total Distance m/2
  Total Distance m underground/1 -> Select Total Distance m/3
  Total Distance m lab_track/1 -> Select Total Distance m/4
  Select Total Distance m/1 -> selectedValue/1

== system HaulageOptimizedOperationSimulation_Bea/Scenario Config/Route Geometry Library/Zone Code Selector ==
  scenarioId : Inport
  Select Zone Code : MultiPortSwitch  SaturateOnIntegerOverflow=off  InputSameDT=off
  Zone Code lab_track : Constant  Value=[1 0 0 0 2 0 0 1]
  Zone Code open_pit : Constant  Value=[1 0 0 0 2 0 0 1]
  Zone Code underground : Constant  Value=[1 0 0 2 0 0 1 1]
  selectedValue : Outport
  wires:
  scenarioId/1 -> [routeScenarioId]
  [routeScenarioId] -> Select Zone Code/1
  Zone Code open_pit/1 -> Select Zone Code/2
  Zone Code underground/1 -> Select Zone Code/3
  Zone Code lab_track/1 -> Select Zone Code/4
  Select Zone Code/1 -> selectedValue/1

== system HaulageOptimizedOperationSimulation_Bea/Scenario Config/Vehicle Truck Specs/Drag Coefficient Selector ==
  scenarioId : Inport
  Drag Coefficient large : Constant  Value=0.7
  Drag Coefficient medium : Constant  Value=0.72
  Drag Coefficient ultra : Constant  Value=0.75
  Select Drag Coefficient : MultiPortSwitch  SaturateOnIntegerOverflow=off  InputSameDT=off
  selectedValue : Outport
  wires:
  scenarioId/1 -> [vehicleScenarioId]
  [vehicleScenarioId] -> Select Drag Coefficient/1
  Drag Coefficient large/1 -> Select Drag Coefficient/2
  Drag Coefficient medium/1 -> Select Drag Coefficient/3
  Drag Coefficient ultra/1 -> Select Drag Coefficient/4
  Select Drag Coefficient/1 -> selectedValue/1

== system HaulageOptimizedOperationSimulation_Bea/Scenario Config/Vehicle Truck Specs/Drivetrain Efficiency Selector ==
  scenarioId : Inport
  Drivetrain Efficiency large : Constant  Value=0.45
  Drivetrain Efficiency medium : Constant  Value=0.46
  Drivetrain Efficiency ultra : Constant  Value=0.43
  Select Drivetrain Efficiency : MultiPortSwitch  SaturateOnIntegerOverflow=off  InputSameDT=off
  selectedValue : Outport
  wires:
  scenarioId/1 -> [vehicleScenarioId]
  [vehicleScenarioId] -> Select Drivetrain Efficiency/1
  Drivetrain Efficiency large/1 -> Select Drivetrain Efficiency/2
  Drivetrain Efficiency medium/1 -> Select Drivetrain Efficiency/3
  Drivetrain Efficiency ultra/1 -> Select Drivetrain Efficiency/4
  Select Drivetrain Efficiency/1 -> selectedValue/1

== system HaulageOptimizedOperationSimulation_Bea/Scenario Config/Vehicle Truck Specs/Empty Mass kg Selector ==
  scenarioId : Inport
  Empty Mass kg large : Constant  Value=150000
  Empty Mass kg medium : Constant  Value=112000
  Empty Mass kg ultra : Constant  Value=250000
  Select Empty Mass kg : MultiPortSwitch  SaturateOnIntegerOverflow=off  InputSameDT=off
  selectedValue : Outport
  wires:
  scenarioId/1 -> [vehicleScenarioId]
  [vehicleScenarioId] -> Select Empty Mass kg/1
  Empty Mass kg large/1 -> Select Empty Mass kg/2
  Empty Mass kg medium/1 -> Select Empty Mass kg/3
  Empty Mass kg ultra/1 -> Select Empty Mass kg/4
  Select Empty Mass kg/1 -> selectedValue/1

== system HaulageOptimizedOperationSimulation_Bea/Scenario Config/Vehicle Truck Specs/Frontal Area m2 Selector ==
  scenarioId : Inport
  Frontal Area m2 large : Constant  Value=10
  Frontal Area m2 medium : Constant  Value=8.5
  Frontal Area m2 ultra : Constant  Value=14
  Select Frontal Area m2 : MultiPortSwitch  SaturateOnIntegerOverflow=off  InputSameDT=off
  selectedValue : Outport
  wires:
  scenarioId/1 -> [vehicleScenarioId]
  [vehicleScenarioId] -> Select Frontal Area m2/1
  Frontal Area m2 large/1 -> Select Frontal Area m2/2
  Frontal Area m2 medium/1 -> Select Frontal Area m2/3
  Frontal Area m2 ultra/1 -> Select Frontal Area m2/4
  Select Frontal Area m2/1 -> selectedValue/1

== system HaulageOptimizedOperationSimulation_Bea/Scenario Config/Vehicle Truck Specs/Idle Fuel Rate Lph Selector ==
  scenarioId : Inport
  Idle Fuel Rate Lph large : Constant  Value=8
  Idle Fuel Rate Lph medium : Constant  Value=7
  Idle Fuel Rate Lph ultra : Constant  Value=12
  Select Idle Fuel Rate Lph : MultiPortSwitch  SaturateOnIntegerOverflow=off  InputSameDT=off
  selectedValue : Outport
  wires:
  scenarioId/1 -> [vehicleScenarioId]
  [vehicleScenarioId] -> Select Idle Fuel Rate Lph/1
  Idle Fuel Rate Lph large/1 -> Select Idle Fuel Rate Lph/2
  Idle Fuel Rate Lph medium/1 -> Select Idle Fuel Rate Lph/3
  Idle Fuel Rate Lph ultra/1 -> Select Idle Fuel Rate Lph/4
  Select Idle Fuel Rate Lph/1 -> selectedValue/1

== system HaulageOptimizedOperationSimulation_Bea/Scenario Config/Vehicle Truck Specs/Max Fuel Rate Lph Selector ==
  scenarioId : Inport
  Max Fuel Rate Lph large : Constant  Value=120
  Max Fuel Rate Lph medium : Constant  Value=95
  Max Fuel Rate Lph ultra : Constant  Value=180
  Select Max Fuel Rate Lph : MultiPortSwitch  SaturateOnIntegerOverflow=off  InputSameDT=off
  selectedValue : Outport
  wires:
  scenarioId/1 -> [vehicleScenarioId]
  [vehicleScenarioId] -> Select Max Fuel Rate Lph/1
  Max Fuel Rate Lph large/1 -> Select Max Fuel Rate Lph/2
  Max Fuel Rate Lph medium/1 -> Select Max Fuel Rate Lph/3
  Max Fuel Rate Lph ultra/1 -> Select Max Fuel Rate Lph/4
  Select Max Fuel Rate Lph/1 -> selectedValue/1

== system HaulageOptimizedOperationSimulation_Bea/Scenario Config/Vehicle Truck Specs/Rated Payload t Selector ==
  scenarioId : Inport
  Rated Payload t large : Constant  Value=279
  Rated Payload t medium : Constant  Value=220
  Rated Payload t ultra : Constant  Value=360
  Select Rated Payload t : MultiPortSwitch  SaturateOnIntegerOverflow=off  InputSameDT=off
  selectedValue : Outport
  wires:
  scenarioId/1 -> [vehicleScenarioId]
  [vehicleScenarioId] -> Select Rated Payload t/1
  Rated Payload t large/1 -> Select Rated Payload t/2
  Rated Payload t medium/1 -> Select Rated Payload t/3
  Rated Payload t ultra/1 -> Select Rated Payload t/4
  Select Rated Payload t/1 -> selectedValue/1

== matlab function HaulageOptimizedOperationSimulation_Bea/Baseline Operation Pipeline/Energy SFC Equations ==
  data: speed_kph input size=1; cumFuel_l output size=1; stepDistance_m input size=1; stepTime_s input size=1; routeVector input size=7; vehicleParams input size=6; fuelRate_lph output size=1; instSfc_l_per_tkm output size=1; productiveTonKm output size=1
function [cumFuel_l, fuelRate_lph, instSfc_l_per_tkm, productiveTonKm] = f(speed_kph, stepDistance_m, stepTime_s, routeVector, vehicleParams)
%#codegen
emptyMass = vehicleParams(1);
idleFuelRate = vehicleParams(2);
maxFuelRate = vehicleParams(3);
frontalArea = vehicleParams(4);
dragCoefficient = vehicleParams(5);
drivetrainEfficiency = vehicleParams(6);
persistent fuel_l prod_tkm
if isempty(fuel_l)
    fuel_l = 0.0;
    prod_tkm = 0.0;
end
effGrade_pct = routeVector(2);
payload_t = routeVector(5);
routeDone = routeVector(7);
fuelRate_lph = idleFuelRate;
instSfc_l_per_tkm = NaN;
cumFuel_l = fuel_l;
productiveTonKm = prod_tkm;
if routeDone < 0.5 && stepTime_s > 0.0
    speed_mps = speed_kph / 3.6;
    g = 9.81;
    rho = 1.225;
    dieselEnergy_kWhPerL = 9.7;
    mass_kg = emptyMass + payload_t * 1000.0;
    gradeForce_N = mass_kg * g * (effGrade_pct / 100.0);
    aeroForce_N = 0.5 * rho * dragCoefficient * frontalArea * speed_mps^2;
    tractiveForce_N = gradeForce_N + aeroForce_N;
    if tractiveForce_N <= 0.0
        fuelRate_lph = idleFuelRate;
    else
        wheelPower_kW = tractiveForce_N * speed_mps / 1000.0;
        fuelRate_lph = idleFuelRate + wheelPower_kW / (drivetrainEfficiency * dieselEnergy_kWhPerL);
    end
    fuelRate_lph = min(max(fuelRate_lph, idleFuelRate), maxFuelRate);
    fuel_l = fuel_l + fuelRate_lph * stepTime_s / 3600.0;
    if payload_t > 0.0
        prod_tkm = prod_tkm + payload_t * stepDistance_m / 1000.0;
        instSfc_l_per_tkm = fuelRate_lph / max(payload_t * speed_kph, eps);
    end
end
cumFuel_l = fuel_l;
productiveTonKm = prod_tkm;

== matlab function HaulageOptimizedOperationSimulation_Bea/Baseline Operation Pipeline/Longitudinal Motion Equations ==
  data: safeSpeed_kph input size=1; speed_kph output size=1; routeVector input size=7; trackingTau_s input size=1; totalRouteDistance input; cumDistance_m output size=1; stepDistance_m output size=1; stepTime_s output size=1
function [speed_kph, cumDistance_m, stepDistance_m, stepTime_s] = f(safeSpeed_kph, routeVector, trackingTau_s, totalRouteDistance)
%#codegen
dt = 1;
persistent speed_mps distance_m
if isempty(speed_mps)
    speed_mps = 0.0;
    distance_m = 0.0;
end
payload_t = routeVector(5);
routeDone = routeVector(7);
speed_kph = speed_mps * 3.6;
cumDistance_m = distance_m;
stepDistance_m = 0.0;
stepTime_s = 0.0;
if routeDone < 0.5
    target_mps = safeSpeed_kph / 3.6;
    if payload_t <= 1.0
        maxAccel = 0.55;
        maxDecel = 0.75;
    elseif payload_t < 225.0
        maxAccel = 0.42;
        maxDecel = 0.68;
    else
        maxAccel = 0.35;
        maxDecel = 0.62;
    end
    speedError = target_mps - speed_mps;
    desiredAccel = speedError / max(trackingTau_s, dt);
    accel = min(max(desiredAccel, -maxDecel), maxAccel);
    speed_mps = max(speed_mps + accel * dt, 0.1);
    remaining_m = max(totalRouteDistance - distance_m, 0.0);
    stepDistance_m = min(speed_mps * dt, remaining_m);
    stepTime_s = stepDistance_m / max(speed_mps, 0.1);
    distance_m = distance_m + stepDistance_m;
end
speed_kph = speed_mps * 3.6;
cumDistance_m = distance_m;

== matlab function HaulageOptimizedOperationSimulation_Bea/Baseline Operation Pipeline/Optimized Speed Advisor/Uphill ==
  data: u input; y output
function y = fcn(u)

if u < 140
    y = 21.255135273793847;

elseif u <= 180
    y = 17.5;

elseif u <= 220
    y = 15.0;

elseif u <= 260
    y = 13.5;

elseif u <= 300
    y = 15.5;
else
    y = 18.5;
end

== matlab function HaulageOptimizedOperationSimulation_Bea/Baseline Operation Pipeline/Optimized Speed Advisor/Flat ==
  data: u input; y output
function y = fcn(u)

if u < 140
    y = 28.362488586323742;

elseif u <= 180
    y = 27.7054122419284;

elseif u <= 220
    y = 27.2374745419987;

elseif u <= 260
    y = 27.335792315325662	;

elseif u <= 300
    y = 27.5;
else
    y = 27.73769876601783;
end

== matlab function HaulageOptimizedOperationSimulation_Bea/Baseline Operation Pipeline/Optimized Speed Advisor/Downhill ==
  data: u input; y output
function y = fcn(u)

if u < 140
    y = 26.3505997741665;

elseif u <= 180
    y = 23.86436991695252;

elseif u <= 220
    y = 22.91079587925706;

elseif u <= 260
    y = 22.0;

elseif u <= 300
    y = 22.5;
else
    y = 24.273372668519478;
end

== matlab function HaulageOptimizedOperationSimulation_Bea/Baseline Results Dashboard and Logs/Baseline Metric Dashboard/Target speed km//h/Uphill ==
  data: u input; y output
function y = fcn(u)

y = u;
